simulink model "lab_03_mdl"  (R2022b)
settings: Solver=FixedStepAuto  StartTime=0.0  StopTime=60  FixedStep=10  RelTol=1e-3
libraries: matrix_library x1
settings Model: Creator=User  LastModifiedBy=User

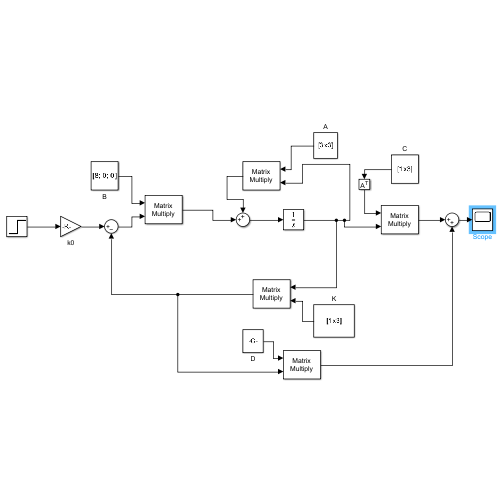
[thumbnail: Simulink's stored preview of the top-level diagram]
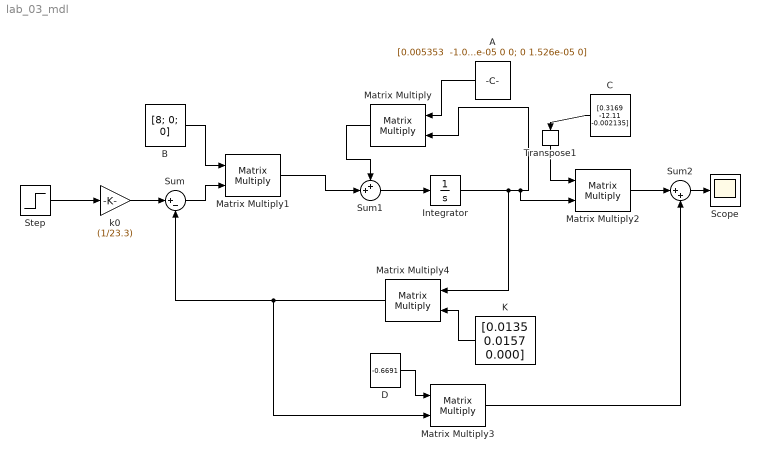
== system lab_03_mdl ==
  A : Constant  Value="[0.005353  -1.029e-05  -1.543e-19; 1.526e-05 0 0; 0 1.526e-05 0]"
  B : Constant  Value=[8; 0; 0]
  C : Constant  Value=[0.3169 -12.11 -0.002135]
  D : Constant  Value=-0.6691
  Integrator : Integrator
  K : Constant  Value="[0.0135    0.0157    0.000]"
  Matrix Multiply{,1..4} (5 alike) : Product  Multiplication=Matrix(*)
  Scope : Scope
  Step : Step  Time=0  SampleTime=0
  Sum : Sum  Inputs=|+-
  Sum1 : Sum  Inputs=++|
  Sum2 : Sum  Inputs=|++
  Transpose1 : matrix_library/Transpose
  k0 : Gain  Gain=(1/23.3)
  wires:
  A/1 -> Matrix Multiply/1
  Matrix Multiply/1 -> Sum1/1
  K/1 -> Matrix Multiply4/2
  Matrix Multiply4/1 -> Matrix Multiply3/2, Sum/2
  Matrix Multiply2/1 -> Sum2/1
  D/1 -> Matrix Multiply3/1
  Sum2/1 -> Scope/1
  B/1 -> Matrix Multiply1/1
  Matrix Multiply1/1 -> Sum1/2
  Sum1/1 -> Integrator/1
  Sum/1 -> Matrix Multiply1/2
  Matrix Multiply3/1 -> Sum2/2
  Integrator/1 -> Matrix Multiply4/1, Matrix Multiply2/2, Matrix Multiply/2
  C/1 -> Transpose1/1
  Transpose1/1 -> Matrix Multiply2/1
  Step/1 -> k0/1
  k0/1 -> Sum/1
